simulink subsystem "TrajectoryExecution"  (R2025b)
settings: Solver=VariableStepAuto  StartTime=0.0  StopTime=10.0  RelTol=1e-3
undefined symbols (not defined in the file): Kp_trajectory, settlingDwell, settlingPositionTol, settlingTimeout, settlingVelocityTol, waypointGoals, waypointTimes
settings Model: Creator=Compu  LastModifiedBy=Compu

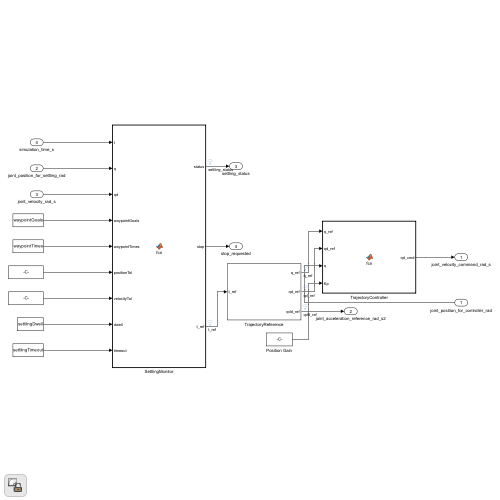
[thumbnail: Simulink's stored preview of the top-level diagram]
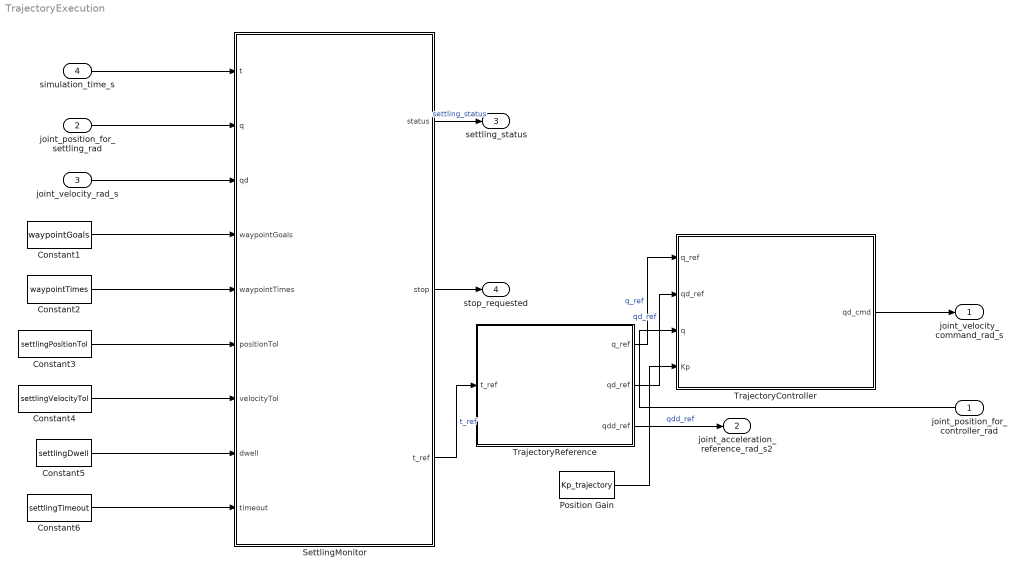
== system TrajectoryExecution ==
  joint_position_for_controller_rad : Inport
  joint_position_for_settling_rad : Inport  Port=2
  joint_velocity_rad_s : Inport  Port=3
  simulation_time_s : Inport  Port=4
  Constant1 : Constant  Value=waypointGoals
  Constant2 : Constant  Value=waypointTimes
  Constant3 : Constant  Value=settlingPositionTol
  Constant4 : Constant  Value=settlingVelocityTol
  Constant5 : Constant  Value=settlingDwell
  Constant6 : Constant  Value=settlingTimeout
  Position Gain : Constant  Value=Kp_trajectory
  SettlingMonitor : MATLAB Function  TreatAsAtomicUnit=on
  TrajectoryController : MATLAB Function  TreatAsAtomicUnit=on
  TrajectoryReference : Subsystem
  joint_velocity_command_rad_s : Outport
  joint_acceleration_reference_rad_s2 : Outport  Port=2
  settling_status : Outport  Port=3
  stop_requested : Outport  Port=4
  wires:
  Position Gain/1 -> TrajectoryController/4(Kp)
  simulation_time_s/1 -> SettlingMonitor/1(t)
  joint_position_for_settling_rad/1 -> SettlingMonitor/2(q)
  joint_velocity_rad_s/1 -> SettlingMonitor/3(qd)
  Constant5/1 -> SettlingMonitor/8(dwell)
  TrajectoryReference/1(q_ref) -> TrajectoryController/1(q_ref)  "q_ref"
  Constant1/1 -> SettlingMonitor/4(waypointGoals)
  Constant3/1 -> SettlingMonitor/6(positionTol)
  Constant2/1 -> SettlingMonitor/5(waypointTimes)
  Constant4/1 -> SettlingMonitor/7(velocityTol)
  Constant6/1 -> SettlingMonitor/9(timeout)
  SettlingMonitor/1(status) -> settling_status/1  "settling_status"
  SettlingMonitor/2(stop) -> stop_requested/1
  SettlingMonitor/3(t_ref) -> TrajectoryReference/1(t_ref)  "t_ref"
  TrajectoryReference/2(qd_ref) -> TrajectoryController/2(qd_ref)  "qd_ref"
  TrajectoryReference/3(qdd_ref) -> joint_acceleration_reference_rad_s2/1  "qdd_ref"
  TrajectoryController/1(qd_cmd) -> joint_velocity_command_rad_s/1
  joint_position_for_controller_rad/1 -> TrajectoryController/3(q)

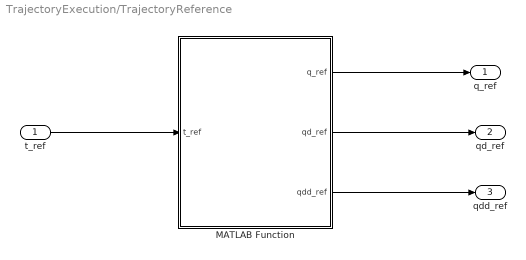
== system TrajectoryExecution/TrajectoryReference ==
  t_ref : Inport
  MATLAB Function : MATLAB Function  TreatAsAtomicUnit=on
  q_ref : Outport
  qd_ref : Outport  Port=2
  qdd_ref : Outport  Port=3
  wires:
  t_ref/1 -> MATLAB Function/1(t_ref)
  MATLAB Function/3(qdd_ref) -> qdd_ref/1
  MATLAB Function/2(qd_ref) -> qd_ref/1
  MATLAB Function/1(q_ref) -> q_ref/1

== matlab function TrajectoryExecution/TrajectoryController ==
  data: q_ref input; qd_cmd output; qd_ref input; q input; Kp input
function qd_cmd = fcn(q_ref, qd_ref, q, Kp)

q_ref  = reshape(q_ref,6,1);
qd_ref = reshape(qd_ref,6,1);
q      = reshape(q,6,1);

positionError = q_ref - q;

qd_cmd = qd_ref + Kp * positionError;

end

== matlab function TrajectoryExecution/SettlingMonitor ==
  data: t input; status output; q input; qd input; waypointGoals input; waypointTimes input; positionTol input; velocityTol input; dwell input; timeout input; stop output; t_ref output
function [status, stop, t_ref] = fcn( ...
    t, q, qd, waypointGoals, waypointTimes, ...
    positionTol, velocityTol, dwell, timeout)

coder.extrinsic('trajectory_segment_info');

persistent segment mode movingStart
persistent settlingStart goodSince refTime

%% 0. Initialize or reset execution

if isempty(mode) || t == 0
    segment = 1;
    mode = 1;
    movingStart = 0;
    settlingStart = 0;
    goodSince = -1;
    refTime = 0;
end

%% 1. Retrieve current trajectory segment

segmentStart = 0;
segmentEnd = 0;
goal = zeros(6,1);
isLast = false;

if mode == 1 || mode == 2

    [segmentStart,segmentEnd,goal,isLast] = ...
        trajectory_segment_info(segment);

end

%% 2. Execute current segment

if mode == 1

    refTime = min(segmentStart + ...
        (t-movingStart), segmentEnd);

    if refTime >= segmentEnd-1e-10
        refTime = segmentEnd;
        mode = 2;
        settlingStart = t;
        goodSince = -1;
    end
end

%% 3. Settle at current waypoint

if mode == 2

    positionError = max(abs(goal-q(:)));
    actualVelocity = max(abs(qd(:)));

    withinTolerance = ...
        positionError <= positionTol && ...
        actualVelocity <= velocityTol;

    if withinTolerance
        if goodSince < 0
            goodSince = t;
        end
    else
        goodSince = -1;
    end

    if goodSince >= 0 && ...
            t-goodSince >= dwell-1e-10

        if isLast
            mode = 3;
        else
            segment = segment + 1;
            movingStart = t;
            goodSince = -1;
            mode = 1;
        end

    elseif t-settlingStart >= timeout-1e-10
        mode = 4;
    end
end

%% 4. Outputs

status = mode;
stop = mode == 3 || mode == 4;
t_ref = refTime;

end

== matlab function TrajectoryExecution/TrajectoryReference/MATLAB Function ==
  data: t_ref input; q_ref output; qd_ref output; qdd_ref output
function [q_ref, qd_ref, qdd_ref] = fcn(t_ref)

coder.extrinsic('evaluate_trajectory_reference');

q_ref   = zeros(6,1);
qd_ref  = zeros(6,1);
qdd_ref = zeros(6,1);

[q_ref, qd_ref, qdd_ref] = ...
    evaluate_trajectory_reference(t_ref);

end
